simulink library "sensors_lib"  (R2018b)
settings: Solver=VariableStepAuto  StartTime=0.0  StopTime=10.0  RelTol=1e-3
settings Model: Creator=Ybeyer  LastModifiedBy=yannic
settings DebuggingCC: LibraryContextMissingDiagnostic=none
settings SFSimCC: SimUseLocalCustomCode=off
settings RTWCC: RTWUseLocalCustomCode=off
settings CodeAppCC: StateflowObjectComments=on

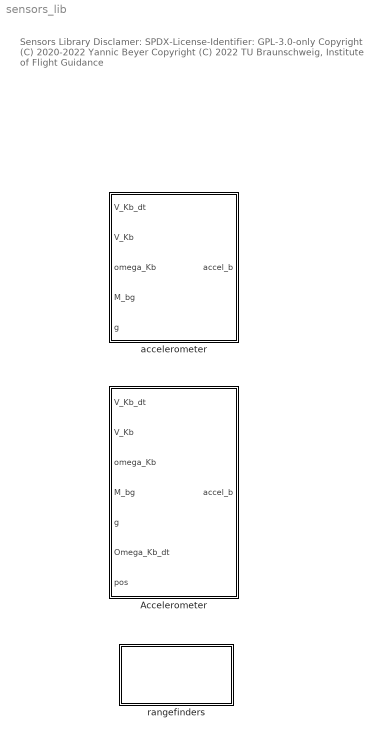
== system sensors_lib ==
  note: Sensors Library
      |
      | Disclamer:
      | SPDX-License-Identifier: GPL-3.0-only
      |
      | Copyright (C) 2020-2022 Yannic Beyer
      | Copyright (C) 2022 TU Braunschweig, Institute of Flight Guidance
  Accelerometer : MATLAB Function  TreatAsAtomicUnit=on
  accelerometer : MATLAB Function  TreatAsAtomicUnit=on
  rangefinders : Subsystem
      settings: OpenFcn=rangefinders_lib

== system sensors_lib/rangefinders ==

== matlab function sensors_lib/Accelerometer ==
  data: V_Kb_dt input; V_Kb input; omega_Kb input; accel_b output; M_bg input; g input; Omega_Kb_dt input; pos input
function accel_b = fcn( V_Kb_dt, V_Kb, omega_Kb, M_bg, g, Omega_Kb_dt, pos ) %#codegen
accel_b = accelerometer( V_Kb_dt, V_Kb, omega_Kb, M_bg, g, Omega_Kb_dt, pos );
end

== matlab function sensors_lib/accelerometer ==
  data: V_Kb_dt input; V_Kb input; omega_Kb input; accel_b output; M_bg input; g input
function accel_b = fcn( V_Kb_dt, V_Kb, omega_Kb, M_bg, g ) %#codegen
accel_b = accelerometer( V_Kb_dt, V_Kb, omega_Kb, M_bg, g );
end
